simulink model "task4_simulation_analytic_jacobian"  (R2025b)
settings: Solver=FixedStepAuto  StartTime=0.0  StopTime=45.4159  RelTol=1e-3
undefined symbols (not defined in the file): d, DiscIntNeverNeededParam, k_theta, k_x, k_y, q_true0, qhat0, r, Ts, X, Y
libraries: robotlib x5
settings Model: Creator=dallaliber  LastModifiedBy=ilia
settings OptimizationCC: DefaultParameterBehavior=Inlined  EnhancedBackFolding=on  PassReuseOutputArgsAs=Individual arguments  ZeroExternalMemoryAtStartup=off  ZeroInternalMemoryAtStartup=off  MaxStackSize=64  OptimizeBlockOrder=speed  DifferentSizesBufferReuse=on  OptimizationCustomize=off  EfficientTunableParamExpr=on
settings DebuggingCC: ParameterTunabilityLossMsg=error
settings HardwareCC: ProdBitPerPointer=32.0  ProdBitPerSizeT=32.0  ProdBitPerPtrDiffT=32.0  ProdLargestAtomicFloat=None  ProdIntDivRoundTo=Undefined  ProdEndianess=Unspecified  ProdWordSize=32.0  ProdHWDeviceType=Generic->Unspecified (assume 32-bit Generic)
settings SFSimCC: MATLABDynamicMemAlloc=off
settings RTWCC: SystemTargetFile=ert.tlc  HardwareBoard=Robot Operating System (ROS)  TLCOptions="-aInlineSetEventsForThisBaseRateFcn=TLC_FALSE -aSuppressMultiTaskScheduler=TLC_FALSE  -aRateBasedStepFcn=0"  TemplateMakefile=ert_default_tmf  Toolchain=Catkin  TargetLang=C++  Description=Embedded Coder
settings CodeAppCC: ForceParamTrailComments=on  IgnoreCustomStorageClasses=off  OperatorAnnotations=on  SimulinkDataObjDesc=on  SFDataObjDesc=on  InsertBlockDesc=on
settings ERTTargetCC: DynamicArrayContainerType=coder::array

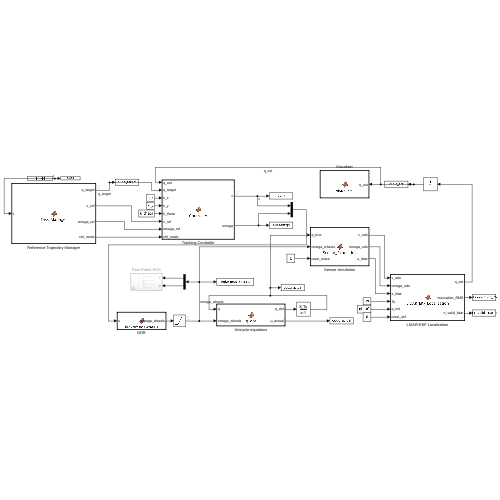
[thumbnail: Simulink's stored preview of the top-level diagram]
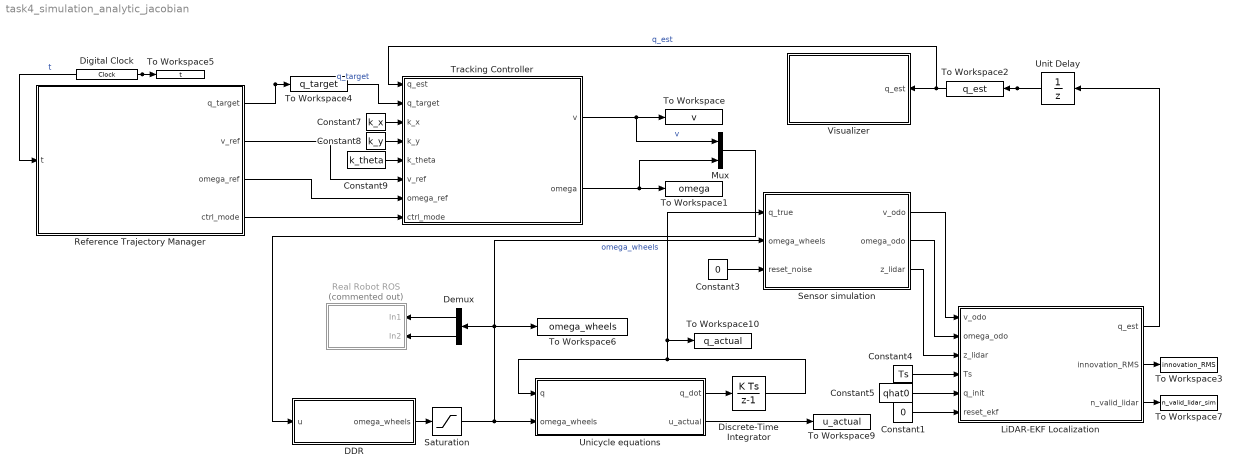
== system task4_simulation_analytic_jacobian ==
  Constant1 : Constant  Value=0
  Constant3 : Constant  Value=0
  Constant4 : Constant  Value=Ts  SampleTime=Ts
  Constant5 : Constant  Value=qhat0  SampleTime=Ts
  Constant7 : Constant  Value=k_x  SampleTime=Ts
  Constant8 : Constant  Value=k_y  SampleTime=Ts
  Constant9 : Constant  Value=k_theta  SampleTime=Ts
  DDR : MATLAB Function  TreatAsAtomicUnit=on
  Demux : Demux  Outputs=2
  Digital Clock : DigitalClock  SampleTime=Ts
  Discrete-Time Integrator : DiscreteIntegrator  InitialCondition=q_true0  SampleTime=Ts  ICPrevOutput=DiscIntNeverNeededParam  ICPrevScaledInput=DiscIntNeverNeededParam
  LiDAR-EKF Localization : MATLAB Function  TreatAsAtomicUnit=on
  Mux : Mux  Inputs=2
  Real Robot ROS : Subsystem  Commented=on
  Reference Trajectory Manager : MATLAB Function  TreatAsAtomicUnit=on
  Saturation : Saturate  UpperLimit=10  LowerLimit=-10
  Sensor simulation : MATLAB Function  TreatAsAtomicUnit=on
  To Workspace : ToWorkspace  VariableName=v  SampleTime=Ts
  To Workspace1 : ToWorkspace  VariableName=omega  SampleTime=Ts
  To Workspace10 : ToWorkspace  VariableName=q_actual  SampleTime=Ts
  To Workspace2 : ToWorkspace  VariableName=q_est  SampleTime=Ts
  To Workspace3 : ToWorkspace  VariableName=innovation_RMS  SampleTime=Ts
  To Workspace4 : ToWorkspace  VariableName=q_target  SampleTime=Ts
  To Workspace5 : ToWorkspace  VariableName=t  SampleTime=Ts
  To Workspace6 : ToWorkspace  VariableName=omega_wheels  SampleTime=Ts
  To Workspace7 : ToWorkspace  VariableName=n_valid_lidar_sim  SampleTime=Ts
  To Workspace9 : ToWorkspace  VariableName=u_actual  SampleTime=Ts
  Tracking Controller : MATLAB Function  TreatAsAtomicUnit=on
  Unicycle equations : MATLAB Function  TreatAsAtomicUnit=on
  Unit Delay : UnitDelay  InitialCondition=qhat0  SampleTime=Ts  HasFrameUpgradeWarning=on
  Visualizer : MATLAB Function  TreatAsAtomicUnit=on
  wires:
  Tracking Controller/1(v) -> To Workspace/1, Mux/1  "v"
  Saturation/1 -> Sensor simulation/2(omega_wheels), To Workspace6/1, Demux/1, Unicycle equations/2(omega_wheels)  "omega_wheels"
  DDR/1(omega_wheels) -> Saturation/1
  Demux/1 -> Real Robot ROS/1(In1)
  Mux/1 -> DDR/1(u)
  Digital Clock/1 -> To Workspace5/1, Reference Trajectory Manager/1(t)  "t"
  Unit Delay/1 -> Tracking Controller/1(q_est), Visualizer/1(q_est), To Workspace2/1  "q_est"
  Tracking Controller/2(omega) -> To Workspace1/1, Mux/2
  Unicycle equations/1(q_dot) -> Discrete-Time Integrator/1
  Discrete-Time Integrator/1 -> To Workspace10/1, Sensor simulation/1(q_true), Unicycle equations/1(q)
  Unicycle equations/2(u_actual) -> To Workspace9/1
  Constant4/1 -> LiDAR-EKF Localization/4(Ts)
  Constant1/1 -> LiDAR-EKF Localization/6(reset_ekf)
  Constant5/1 -> LiDAR-EKF Localization/5(q_init)
  LiDAR-EKF Localization/1(q_est) -> Unit Delay/1
  Demux/2 -> Real Robot ROS/2(In2)
  Sensor simulation/3(z_lidar) -> LiDAR-EKF Localization/3(z_lidar)
  Sensor simulation/2(omega_odo) -> LiDAR-EKF Localization/2(omega_odo)
  Sensor simulation/1(v_odo) -> LiDAR-EKF Localization/1(v_odo)
  Constant3/1 -> Sensor simulation/3(reset_noise)
  Constant8/1 -> Tracking Controller/4(k_y)
  Constant7/1 -> Tracking Controller/3(k_x)
  Constant9/1 -> Tracking Controller/5(k_theta)
  Reference Trajectory Manager/1(q_target) -> To Workspace4/1, Tracking Controller/2(q_target)  "q_target"
  Reference Trajectory Manager/2(v_ref) -> Tracking Controller/6(v_ref)
  Reference Trajectory Manager/3(omega_ref) -> Tracking Controller/7(omega_ref)
  Reference Trajectory Manager/4(ctrl_mode) -> Tracking Controller/8(ctrl_mode)
  LiDAR-EKF Localization/2(innovation_RMS) -> To Workspace3/1
  LiDAR-EKF Localization/3(n_valid_lidar) -> To Workspace7/1

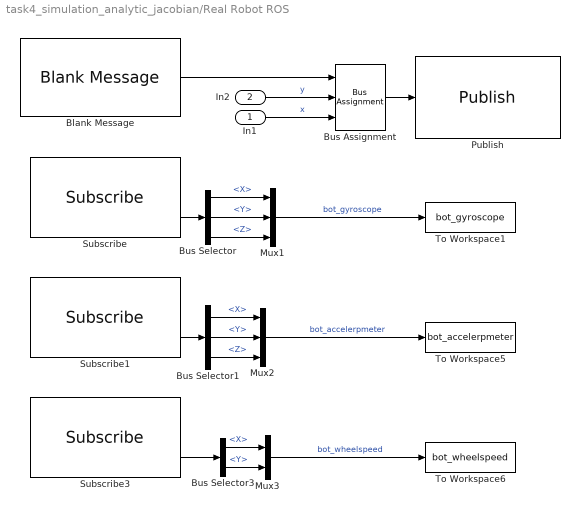
== system task4_simulation_analytic_jacobian/Real Robot ROS ==
  In1 : Inport
  In2 : Inport  Port=2
  Blank Message : robotlib/Blank Message  messageClass=Message  entityType=geometry_msgs/Vector3  messageType=geometry_msgs/Vector3  SampleTime=0.04  legacyBusStruct=off
  Bus Assignment : BusAssignment  AssignedSignals=X,Y
  Bus Selector : BusSelector  OutputSignals=X,Y,Z
  Bus Selector1 : BusSelector  OutputSignals=X,Y,Z
  Bus Selector3 : BusSelector  OutputSignals=X,Y
  Mux1 : Mux  Inputs=3
  Mux2 : Mux  Inputs=3
  Mux3 : Mux  Inputs=2
  Publish : robotlib/Publish  topicSource=Select from ROS network  topic=/turtlebot_09/cmd_wheels  messageType=geometry_msgs/Vector3  legacyBusStruct=off  messageQueueLength=1
  Subscribe : robotlib/Subscribe  topicSource=Select from ROS network  topic=/turtlebot_09/gyroscope  messageType=geometry_msgs/Vector3  SampleTime=0.04  legacyBusStruct=off  messageQueueLength=1
  Subscribe1 : robotlib/Subscribe  topicSource=Select from ROS network  topic=/turtlebot_09/accelerometer  messageType=geometry_msgs/Vector3  SampleTime=0.04  legacyBusStruct=off  messageQueueLength=1
  Subscribe3 : robotlib/Subscribe  topicSource=Select from ROS network  topic=/turtlebot_09/wheelSpeeds  messageType=geometry_msgs/Vector3  SampleTime=0.04  legacyBusStruct=off  messageQueueLength=1
  To Workspace1 : ToWorkspace  VariableName=bot_gyroscope  SaveFormat=Timeseries  SampleTime=Ts
  To Workspace5 : ToWorkspace  VariableName=bot_accelerpmeter  SaveFormat=Timeseries  SampleTime=Ts
  To Workspace6 : ToWorkspace  VariableName=bot_wheelspeed  SaveFormat=Timeseries  SampleTime=Ts
  wires:
  Subscribe1/2 -> Bus Selector1/1
  Bus Selector1/1 -> Mux2/1  "<X>"
  Mux2/1 -> To Workspace5/1  "bot_accelerpmeter"
  Bus Assignment/1 -> Publish/1
  Subscribe/2 -> Bus Selector/1
  Bus Selector/2 -> Mux1/2  "<Y>"
  Bus Selector/1 -> Mux1/1  "<X>"
  Bus Selector3/1 -> Mux3/1  "<X>"
  Bus Selector3/2 -> Mux3/2  "<Y>"
  Bus Selector1/3 -> Mux2/3  "<Z>"
  Bus Selector1/2 -> Mux2/2  "<Y>"
  Mux3/1 -> To Workspace6/1  "bot_wheelspeed"
  Mux1/1 -> To Workspace1/1  "bot_gyroscope"
  Subscribe3/2 -> Bus Selector3/1
  Blank Message/1 -> Bus Assignment/1
  Bus Selector/3 -> Mux1/3  "<Z>"
  In1/1 -> Bus Assignment/3  "x"
  In2/1 -> Bus Assignment/2  "y"

== matlab function task4_simulation_analytic_jacobian/Tracking Controller ==
  data: q_est input; q_target input; v output; k_x input; omega output; k_y input; k_theta input; v_ref input; omega_ref input; ctrl_mode input
function [v, omega] = Controller(q_est, q_target, k_x, k_y, k_theta, v_ref, omega_ref, ctrl_mode)
%#codegen
% Tracking Controller
% ctrl_mode = 1: approach/regulation
% ctrl_mode = 2: trajectory tracking
% ctrl_mode = 3: stop

theta = q_est(3);

dx = q_target(1) - q_est(1);
dy = q_target(2) - q_est(2);

dtheta = wrapToPiLocal(q_target(3) - q_est(3));

%% Limits
v_lim = 0.22;
omega_lim = 0.80;

%% Mode 2: trajectory tracking
if ctrl_mode == 2

    ex =  cos(theta)*dx + sin(theta)*dy;
    ey = -sin(theta)*dx + cos(theta)*dy;
    eth = dtheta;

    k1 = 0.75;
    k2 = 2.00;
    k3 = 1.20;

    v = v_ref*cos(eth) + k1*ex;
    omega = omega_ref + k2*v_ref*ey + k3*sin(eth);

%% Mode 1: approach to circle start
elseif ctrl_mode == 1

    rho = sqrt(dx^2 + dy^2);
    angle_to_goal = atan2(dy, dx);
    alpha = wrapToPiLocal(angle_to_goal - theta);

    k_rho = 0.55;
    k_alpha = 1.20;
    k_final = 0.95;

    rho_switch = 0.010;

    if rho > rho_switch

        v = k_rho*rho*cos(alpha);

        if abs(alpha) > 1.2
            v = 0.0;
        elseif abs(alpha) > 0.6
            v = 0.4*v;
        end

        omega = k_alpha*alpha;

    else

        v = 0.0;
        omega = k_final*dtheta;

    end

%% Mode 3: stop
else

    v = 0.0;
    omega = 0.0;

end

%% Saturation
v = satLocal(v, -v_lim, v_lim);
omega = satLocal(omega, -omega_lim, omega_lim);

end

function y = satLocal(u, umin, umax)
y = min(max(u, umin), umax);
end

function a = wrapToPiLocal(a)
a = atan2(sin(a), cos(a));
end

== matlab function task4_simulation_analytic_jacobian/Visualizer ==
  data: q_est input
function visualizer(q_est)
    coder.extrinsic('draw_robot');
    draw_robot(q_est(1), q_est(2));
end

== matlab function task4_simulation_analytic_jacobian/LiDAR-EKF Localization ==
  data: v_odo input; omega_odo input; z_lidar input; Ts input; q_est output; q_init input; reset_ekf input; innovation_RMS output; n_valid_lidar output
function [q_est, innovation_RMS, n_valid_lidar] = fcn(v_odo, omega_odo, z_lidar, Ts, q_init, reset_ekf)
% LiDAR_EKF_Localization
%
% EKF localization for Task 4 using:
% - odometry / IMU prediction
% - analytical LiDAR ray-wall Jacobian
%
% Inputs:
%   v_odo      : odometric linear velocity [m/s]
%   omega_odo  : odometric angular velocity [rad/s]
%   z_lidar    : simulated LiDAR ranges, 36x1 [m]
%   Ts         : sampling time [s]
%   q_init     : EKF initial estimate, 3x1
%   reset_ekf  : reset flag
%
% Outputs:
%   q_est          : estimated pose, 3x1
%   innovation_RMS : RMS innovation after gating [m]
%   n_valid_lidar  : number of LiDAR beams used in EKF update

%#codegen

persistent q_hat P k_counter

%% ============================================================
%  Fixed Task 4 EKF parameters
% ============================================================

% Nominal initial pose used only to select exact/wrong-EKF tuning.
q_nominal = [0.960; -0.340; deg2radLocal(4.00)];

% Process covariance
Q = diag([1.5e-5, 1.5e-5, 6e-5]);

% LiDAR geometry
Nbeams = 36;
lidar_offset = 0.076;

% Known cube geometry
cube_x_min = 1.80;
cube_x_max = 2.20;
cube_y_min = -0.20;
cube_y_max = 0.20;

% Decide whether this is exact initialization or wrong-EKF initialization.
% In exact case:
%   q_init = q_true0 = q_nominal
% In wrong-EKF case:
%   q_init = qhat0 ~= q_true0
init_difference_pos = sqrt((q_init(1)-q_nominal(1))^2 + (q_init(2)-q_nominal(2))^2);
init_difference_th  = abs(wrapPiLocal(q_init(3)-q_nominal(3)));

wrong_ekf_initialization = (init_difference_pos > 0.02) || (init_difference_th > deg2radLocal(2.0));

if wrong_ekf_initialization
    P0 = diag([5e-3, 5e-3, deg2radLocal(7)^2]);
    gate_initial = 0.120;
    gate_after   = 0.080;
    min_valid_required = 3;
    R_lidar_scalar = (0.006)^2;
else
    P0 = diag([1e-4, 1e-4, deg2radLocal(1)^2]);
    gate_initial = 0.045;
    gate_after   = 0.045;
    min_valid_required = 4;
    R_lidar_scalar = (0.010)^2;
end

%% ============================================================
%  Initialize / reset EKF
% ============================================================

if isempty(q_hat) || isempty(P) || isempty(k_counter) || reset_ekf ~= 0
    q_hat = q_init;
    q_hat(3) = wrapPiLocal(q_hat(3));

    P = P0;
    k_counter = 0;
end

k_counter = k_counter + 1;

%% ============================================================
%  EKF prediction step
% ============================================================

theta = q_hat(3);

theta_mid = theta + 0.5*Ts*omega_odo;

q_pred = zeros(3,1);
q_pred(1) = q_hat(1) + Ts*v_odo*cos(theta_mid);
q_pred(2) = q_hat(2) + Ts*v_odo*sin(theta_mid);
q_pred(3) = wrapPiLocal(q_hat(3) + Ts*omega_odo);

F = eye(3);
F(1,3) = -Ts*v_odo*sin(theta_mid);
F(2,3) =  Ts*v_odo*cos(theta_mid);

P_pred = F*P*F' + Q;

%% ============================================================
%  Analytical LiDAR prediction and Jacobian
% ============================================================

[z_hat_all, H_all, valid_pred] = lidarModelAnalytic( ...
    q_pred, ...
    Nbeams, ...
    lidar_offset, ...
    cube_x_min, cube_x_max, ...
    cube_y_min, cube_y_max);

%% ============================================================
%  Innovation gating
% ============================================================

if k_counter <= round(3.0/Ts)
    lidar_gate = gate_initial;
else
    lidar_gate = gate_after;
end

innov_stack = zeros(Nbeams,1);
H_stack = zeros(Nbeams,3);

count = 0;

for i = 1:Nbeams

    zi = z_lidar(i);

    z_is_valid = isfiniteLocal(zi) && (zi > 0);

    if z_is_valid && valid_pred(i)

        innov_i = zi - z_hat_all(i);

        if abs(innov_i) <= lidar_gate

            count = count + 1;

            innov_stack(count) = innov_i;
            H_stack(count,:) = H_all(i,:);

        end
    end
end

n_valid_lidar = count;

%% ============================================================
%  EKF correction step
% ============================================================

q_upd = q_pred;
P_upd = P_pred;

if count >= min_valid_required

    sumInnov2 = 0;

    for j = 1:count

        Hrow = H_stack(j,:);       % 1x3
        innov = innov_stack(j);    % scalar

        S = Hrow*P_upd*Hrow' + R_lidar_scalar;

        if S > 1e-12

            K = (P_upd*Hrow')/S;   % 3x1

            q_upd = q_upd + K*innov;
            q_upd(3) = wrapPiLocal(q_upd(3));

            % Joseph-stabilized covariance update for scalar measurement
            I3 = eye(3);
            KH = K*Hrow;
            P_upd = (I3 - KH)*P_upd*(I3 - KH)' + K*R_lidar_scalar*K';

            sumInnov2 = sumInnov2 + innov^2;
        end
    end

    innovation_RMS = sqrt(sumInnov2 / count);

else

    % Not enough valid LiDAR beams: prediction only
    innovation_RMS = NaN;

end

%% ============================================================
%  Save persistent state and output
% ============================================================

q_hat = q_upd;
P = P_upd;

q_est = q_hat;

end

%% ========================================================================
%  Analytical LiDAR model and Jacobian
% ========================================================================

function [z_pred, H_all, valid_pred] = lidarModelAnalytic(q, Nbeams, l, cube_x_min, cube_x_max, cube_y_min, cube_y_max)
% Analytical LiDAR range model and Jacobian for a known square cube.
%
% For each beam, the function checks the four cube walls and selects the
% nearest positive valid ray-wall intersection.

z_pred = NaN(Nbeams,1);
H_all = zeros(Nbeams,3);
valid_pred = false(Nbeams,1);

x = q(1);
y = q(2);
th = q(3);

px = x + l*cos(th);
py = y + l*sin(th);

for i = 1:Nbeams

    theta_i = -pi + (i-1)*(2*pi/Nbeams);
    phi = th + theta_i;

    best_h = inf;
    best_H = zeros(1,3);
    best_valid = false;

    %% Wall 1: x = cube_x_min
    [h, Hrow, ok] = rayLineJacobian(q, theta_i, 1, 0, -cube_x_min, l);
    if ok
        Xint = px + h*cos(phi);
        Yint = py + h*sin(phi);

        if isInside(Yint, cube_y_min, cube_y_max) && h < best_h
            best_h = h;
            best_H = Hrow;
            best_valid = true;
        end
    end

    %% Wall 2: x = cube_x_max
    [h, Hrow, ok] = rayLineJacobian(q, theta_i, 1, 0, -cube_x_max, l);
    if ok
        Xint = px + h*cos(phi);
        Yint = py + h*sin(phi);

        if isInside(Yint, cube_y_min, cube_y_max) && h < best_h
            best_h = h;
            best_H = Hrow;
            best_valid = true;
        end
    end

    %% Wall 3: y = cube_y_min
    [h, Hrow, ok] = rayLineJacobian(q, theta_i, 0, 1, -cube_y_min, l);
    if ok
        Xint = px + h*cos(phi);
        Yint = py + h*sin(phi);

        if isInside(Xint, cube_x_min, cube_x_max) && h < best_h
            best_h = h;
            best_H = Hrow;
            best_valid = true;
        end
    end

    %% Wall 4: y = cube_y_max
    [h, Hrow, ok] = rayLineJacobian(q, theta_i, 0, 1, -cube_y_max, l);
    if ok
        Xint = px + h*cos(phi);
        Yint = py + h*sin(phi);

        if isInside(Xint, cube_x_min, cube_x_max) && h < best_h
            best_h = h;
            best_H = Hrow;
            best_valid = true;
        end
    end

    if best_valid
        z_pred(i) = best_h;
        H_all(i,:) = best_H;
        valid_pred(i) = true;
    end
end

end

%% ========================================================================
%  Analytical ray-line Jacobian
% ========================================================================

function [h, Hrow, valid] = rayLineJacobian(q, theta_i, A, B, C, l)
% Analytical ray-line intersection range and Jacobian.
%
% Wall:
%   A X + B Y + C = 0
%
% Ray:
%   p(s) = p_L + s [cos(phi); sin(phi)]
%
% Predicted range:
%   h = -N/D

x = q(1);
y = q(2);
th = q(3);

px = x + l*cos(th);
py = y + l*sin(th);

phi = th + theta_i;

N = A*px + B*py + C;
D = A*cos(phi) + B*sin(phi);

h = NaN;
Hrow = zeros(1,3);
valid = false;

if abs(D) < 1e-9
    return;
end

h = -N/D;

if h <= 0
    return;
end

dN_dtheta = l*(-A*sin(th) + B*cos(th));
dD_dtheta = -A*sin(phi) + B*cos(phi);

dh_dx = -A/D;
dh_dy = -B/D;
dh_dtheta = (N*dD_dtheta - dN_dtheta*D)/(D^2);

Hrow(1) = dh_dx;
Hrow(2) = dh_dy;
Hrow(3) = dh_dtheta;

valid = true;

end

%% ========================================================================
%  Utility functions
% ========================================================================

function ok = isInside(value, lowerBound, upperBound)

tol = 1e-9;
ok = (value >= lowerBound - tol) && (value <= upperBound + tol);

end

function a = wrapPiLocal(a)

a = atan2(sin(a), cos(a));

end

function r = deg2radLocal(d)

r = d*pi/180;

end

function tf = isfiniteLocal(x)

tf = ~isnan(x) && ~isinf(x);

end

== matlab function task4_simulation_analytic_jacobian/DDR ==
  data: u input; omega_wheels output; r parameter; d parameter
function omega_wheels = kin2omegawheels(u, r, d)
omega_l = u(1)/r-d/(2*r)*u(2);
omega_r = u(1)/r+d/(2*r)*u(2);
omega_wheels = [omega_l;omega_r];

== matlab function task4_simulation_analytic_jacobian/Unicycle equations ==
  data: q input; omega_wheels input; q_dot output; r parameter; d parameter; u_actual output
function [q_dot, u_actual] = q_dot(q, omega_wheels, r, d)
u_actual = [r/2, r/2;-r/d, r/d]*omega_wheels;
theta = q(3);
q_dot = [[cos(theta), 0];[sin(theta), 0];[0,1]]*u_actual;

== matlab function task4_simulation_analytic_jacobian/Reference Trajectory Manager ==
  data: t input; q_target output; v_ref output; omega_ref output; ctrl_mode output
function [q_target, v_ref, omega_ref, ctrl_mode] = Task_Manager(t)
%#codegen
% Reference Trajectory Manager for Task 4
% Phase 1: Hermite approach trajectory
% Phase 2: circular trajectory around the cube
% Phase 3: stop / hold final pose

%% ============================================================
% Geometry and timing
% ============================================================

% Initial true pose, close to the final configuration of Task 2
q0 = [0.96; -0.34; 4*pi/180];

% Circle start point
x_start = 1.45;
y_start = -0.30;

% Cube / circle center
xc = 2.00;
yc = 0.00;

dx0 = x_start - xc;
dy0 = y_start - yc;

R_circle = sqrt(dx0^2 + dy0^2);

circle_dir = 1.0;
omega_circle_abs = 0.30;      % [rad/s]

N_turns = 1.5;
T_circle = 2*pi*N_turns/omega_circle_abs;

T_approach = 8.0;             % [s]

alpha0 = atan2(dy0, dx0);
theta_start = wrapToPiLocal(alpha0 + circle_dir*pi/2);

q_start = [x_start; y_start; theta_start];

%% Default outputs

q_target = zeros(3,1);
v_ref = 0.0;
omega_ref = 0.0;
ctrl_mode = 2.0;

%% ============================================================
% Phase 1: Hermite approach trajectory
% ============================================================

if t < T_approach

    tau = t/T_approach;

    if tau < 0
        tau = 0;
    elseif tau > 1
        tau = 1;
    end

    % Smooth time law
    s = 10*tau^3 - 15*tau^4 + 6*tau^5;
    sdot = (30*tau^2 - 60*tau^3 + 30*tau^4)/T_approach;
    sddot = (60*tau - 180*tau^2 + 120*tau^3)/(T_approach^2);

    % Hermite geometry
    p0 = q0(1:2);
    p1 = q_start(1:2);

    L = norm(p1 - p0);

    if L < 0.45
        L = 0.45;
    end

    m0 = L*[cos(q0(3)); sin(q0(3))];
    m1 = L*[cos(q_start(3)); sin(q_start(3))];

    h00 =  2*s^3 - 3*s^2 + 1;
    h10 =      s^3 - 2*s^2 + s;
    h01 = -2*s^3 + 3*s^2;
    h11 =      s^3 -   s^2;

    dh00 =  6*s^2 - 6*s;
    dh10 =  3*s^2 - 4*s + 1;
    dh01 = -6*s^2 + 6*s;
    dh11 =  3*s^2 - 2*s;

    d2h00 =  12*s - 6;
    d2h10 =   6*s - 4;
    d2h01 = -12*s + 6;
    d2h11 =   6*s - 2;

    p = h00*p0 + h10*m0 + h01*p1 + h11*m1;

    dpds = dh00*p0 + dh10*m0 + dh01*p1 + dh11*m1;
    d2pds2 = d2h00*p0 + d2h10*m0 + d2h01*p1 + d2h11*m1;

    pdot = dpds*sdot;
    pddot = d2pds2*(sdot^2) + dpds*sddot;

    v_ref = sqrt(pdot(1)^2 + pdot(2)^2);

    if v_ref > 1e-5

        theta_ref = atan2(pdot(2), pdot(1));

        omega_ref = (pdot(1)*pddot(2) - pdot(2)*pddot(1))/(v_ref^2);

    else

        if tau < 0.5
            theta_ref = q0(3);
        else
            theta_ref = q_start(3);
        end

        omega_ref = 0.0;

    end

    % Avoid unrealistic angular feedforward during very slow motion
    omega_ref = satLocal(omega_ref, -0.80, 0.80);

    q_target = [p(1); p(2); wrapToPiLocal(theta_ref)];

    ctrl_mode = 2.0;

%% ============================================================
% Phase 2: circular trajectory tracking
% ============================================================

elseif t < T_approach + T_circle

    elapsed_circle = t - T_approach;

    alpha = alpha0 + circle_dir*omega_circle_abs*elapsed_circle;

    xd = xc + R_circle*cos(alpha);
    yd = yc + R_circle*sin(alpha);
    thd = wrapToPiLocal(alpha + circle_dir*pi/2);

    q_target = [xd; yd; thd];

    v_ref = R_circle*omega_circle_abs;
    omega_ref = circle_dir*omega_circle_abs;

    ctrl_mode = 2.0;

%% ============================================================
% Phase 3: stop / hold final pose
% ============================================================

else

    alpha = alpha0 + circle_dir*omega_circle_abs*T_circle;

    xd = xc + R_circle*cos(alpha);
    yd = yc + R_circle*sin(alpha);
    thd = wrapToPiLocal(alpha + circle_dir*pi/2);

    q_target = [xd; yd; thd];

    v_ref = 0.0;
    omega_ref = 0.0;

    ctrl_mode = 3.0;

end

end

function y = satLocal(u, umin, umax)

y = min(max(u, umin), umax);

end

function a = wrapToPiLocal(a)

a = atan2(sin(a), cos(a));

end

== matlab function task4_simulation_analytic_jacobian/Sensor simulation ==
  data: q_true input; v_odo output; omega_wheels input; reset_noise input; omega_odo output; z_lidar output
function [v_odo, omega_odo, z_lidar] = Sensor_Simulation(q_true, omega_wheels, reset_noise)
%#codegen
% Simulated encoders, IMU yaw-rate, and LiDAR range measurements

persistent seed

if isempty(seed) || reset_noise > 0.5
    seed = 123456789.0;
end

%% Robot parameters
Ts = 0.04;
r = 0.03;
d = 0.165;

%% Artificial simulation perturbations
sigma_encoder = 0.0008;   % [rad]
sigma_imu_w   = 0.010;    % [rad/s]
sigma_lidar   = 0.006;    % [m]
p_dropout     = 0.03;

%% Wheel encoder / IMU simulation
omega_L = omega_wheels(1);
omega_R = omega_wheels(2);

[n1, seed] = gaussianLCG(seed);
[n2, seed] = gaussianLCG(seed);

dphiL = omega_L*Ts + sigma_encoder*n1;
dphiR = omega_R*Ts + sigma_encoder*n2;

v_enc = r*(dphiL + dphiR)/(2*Ts);
omega_enc = r*(dphiR - dphiL)/(d*Ts);

omega_true = r*(omega_R - omega_L)/d;

[n3, seed] = gaussianLCG(seed);
omega_imu = omega_true + sigma_imu_w*n3;

v_odo = v_enc;
omega_odo = 0.45*omega_enc + 0.55*omega_imu;

%% LiDAR simulation
z_clean = lidarModel(q_true);

z_lidar = zeros(36,1);

for i = 1:36

    if isfinite(z_clean(i))

        [n, seed] = gaussianLCG(seed);
        [u, seed] = uniformLCG(seed);

        if u < p_dropout
            z_lidar(i) = NaN;
        else
            z_lidar(i) = z_clean(i) + sigma_lidar*n;

            if z_lidar(i) < 0.02
                z_lidar(i) = 0.02;
            end
        end

    else

        z_lidar(i) = NaN;

    end

end

end

%% ============================================================
% LiDAR model
% ============================================================
function h = lidarModel(q)

lidar_offset = 0.076;

x = q(1);
y = q(2);
theta = q(3);

pL = [x; y] + lidar_offset*[cos(theta); sin(theta)];

h = NaN(36,1);

for i = 1:36

    angle_rel = -pi + (i-1)*(2*pi/36);
    alpha = theta + angle_rel;

    h(i) = rayBoxDistance(pL, alpha);

end

end

function dist = rayBoxDistance(p, alpha)

cube_xmin = 1.80;
cube_xmax = 2.20;
cube_ymin = -0.20;
cube_ymax = 0.20;

lidar_max_range = 3.0;

dir = [cos(alpha); sin(alpha)];

best = 1e9;
found = false;

%% Vertical walls
if abs(dir(1)) > 1e-10

    tx1 = (cube_xmin - p(1))/dir(1);
    yx1 = p(2) + tx1*dir(2);

    if tx1 > 1e-6 && yx1 >= cube_ymin && yx1 <= cube_ymax
        best = min(best, tx1);
        found = true;
    end

    tx2 = (cube_xmax - p(1))/dir(1);
    yx2 = p(2) + tx2*dir(2);

    if tx2 > 1e-6 && yx2 >= cube_ymin && yx2 <= cube_ymax
        best = min(best, tx2);
        found = true;
    end

end

%% Horizontal walls
if abs(dir(2)) > 1e-10

    ty1 = (cube_ymin - p(2))/dir(2);
    xy1 = p(1) + ty1*dir(1);

    if ty1 > 1e-6 && xy1 >= cube_xmin && xy1 <= cube_xmax
        best = min(best, ty1);
        found = true;
    end

    ty2 = (cube_ymax - p(2))/dir(2);
    xy2 = p(1) + ty2*dir(1);

    if ty2 > 1e-6 && xy2 >= cube_xmin && xy2 <= cube_xmax
        best = min(best, ty2);
        found = true;
    end

end

if found && best <= lidar_max_range
    dist = best;
else
    dist = NaN;
end

end

%% ============================================================
% Random generators
% ============================================================
function [u, seed] = uniformLCG(seed)

a = 1664525.0;
c = 1013904223.0;
m = 4294967296.0;

seed = mod(a*seed + c, m);
u = (seed + 1.0)/(m + 2.0);

end

function [z, seed] = gaussianLCG(seed)

[u1, seed] = uniformLCG(seed);
[u2, seed] = uniformLCG(seed);

if u1 < 1e-12
    u1 = 1e-12;
end

z = sqrt(-2.0*log(u1))*cos(2.0*pi*u2);

end
